simulink model "TestModel_V5_Timing_V3_2024a"  (R2024a)
settings: Solver=FixedStepAuto  StartTime=0.0  StopTime=40  FixedStep=1e-6  RelTol=1e-3
values from neighbouring files (symbols this model uses):
  par_Ctrl_FluxOffset = 0    [Param.m]
  par_Ctrl_MI = 0.99    [Param.m]
  par_Ctrl_SpdRt = 10    [Param.m]
  par_Ctrl_ThetaOffset = 0    [Param.m]
  par_IM_Frated = 50    [Param.m]
  par_IM_IratedPh = 7.9/sqrt(3)    [Param.m]
  par_IM_Lm = 0.527    [Param.m]
  par_IM_Lr = par_IM_Lm + par_IM_Llr    (= 0.5639)    [Param.m]
  par_IM_pp = 2    [Param.m]
  par_IM_Rs = 3.14    [Param.m]
  par_IM_VrmsLL = 400    [Param.m]
  par_uc_Ts = 100e-6    (= 0.0001)    [Param.m]
  pmsm = mcb.getPMSMParameters('Teknic2310P')    [mcb_pmsm_foc_sensorless_f28379d_datascript.m]
  Ts = T_pwm    (= 5e-05)    [mcb_pmsm_foc_sensorless_f28379d_datascript.m]
  Ts_motor = T_pwm/2    (= 2.5e-05)    [mcb_pmsm_foc_sensorless_f28379d_datascript.m]
undefined symbols (not defined in the file or in its folder): DiscIntNeverNeededParam, IM, par_pmsm_FluxLinkage, par_pmsm_Frated, par_pmsm_pp, par_pmsm_Vboost, par_pmsm_VrmsLL
libraries: spsOnDelayLib x24, mcbcontrolslib x12, spsTriangleGeneratorLib x4, autolibim x3, spsFirstOrderFilterLib x3, spsCurrentMeasurementLib x2, spsDCVoltageSourceLib x2, spsVoltageMeasurementLib x2, spsTwoLevelConverterLib x2, spsThreePhaseVIMeasurementLib x2, spsSeriesRLCBranchLib x1, sdolib x1
(part 3 of 3)

== matlab function TestModel_V5_Timing_V3_2024a/Open_Loop2/Estimation/MRAS_Observer ==
  data: v_alpha input; theta_est output; v_beta input; i_alpha input; i_beta input; Ts input; Rs input; Rr input; Ls input; Lr input; Lm input; Kp_SpdEst input; Ki_SpdEst input; omega_est output; e output; e_filt output; psi_r_ref_alpha output; psi_r_ref_beta output; psi_r_est_alpha1 output; psi_r_est_beta1 output; psi_est_mag1 output; psi_ref_mag1 output; psi_s_alpha1 output; psi_s_beta1 output; psi_mag_stator1 output; psi_r_est_alpha_dot1 output; psi_r_est_beta_dot1 output; Fe_Out input
function [theta_est, omega_est, e, e_filt, psi_r_ref_alpha, psi_r_ref_beta, psi_r_est_alpha1, psi_r_est_beta1, psi_est_mag1, psi_ref_mag1, psi_s_alpha1, psi_s_beta1, psi_mag_stator1, psi_r_est_alpha_dot1, psi_r_est_beta_dot1] = fcn(v_alpha, v_beta, i_alpha, i_beta, Ts, Rs, Rr, Ls, Lr, Lm, Kp_SpdEst, Ki_SpdEst, Fe_Out)

%% Motor Parameters

Tr = Lr/Rr;   % Rotor time constant
sigma = 1 - (Lm^2)/(Ls*Lr);

%% Flux Integrator Leakage Factor

wc_flux = 20;      % rad/s

%% Speed LPF Bandwidth

wc_speed = 100;   % rad/s

%% Limits

INT_LIMIT = 500;

OMEGA_MAX = 1000;
OMEGA_MIN = -1000;

FLUX_MIN = 0;
%FLUX_MIN = 0.05;

%% Persistent Variables

persistent psi_s_alpha psi_s_beta

persistent psi_r_est_alpha psi_r_est_beta

persistent omega_hat
persistent omega_filt

persistent theta_hat

persistent int_error
% persistent e_prev

if isempty(psi_s_alpha)

    psi_s_alpha = 0;
    psi_s_beta = 0;

    psi_r_est_alpha = 0;
    psi_r_est_beta = 0;

    omega_hat = 1;   % Small non-zero initial value
    omega_filt = 100;

    theta_hat = 0;

    int_error = 0;
    % e_prev = 0;

end

persistent e_filt_prv

if isempty(e_filt_prv)
    e_filt_prv = 0;
end

% if isempty(int_error)
%     int_error = 0;
% end


%% ==========================================================
%% REFERENCE MODEL
%% Voltage Model
%% ==========================================================

psi_s_alpha_dot = v_alpha - Rs*i_alpha;
psi_s_beta_dot  = v_beta  - Rs*i_beta;

% Leaky Integrator

psi_s_alpha = ...
    (1 - wc_flux*Ts)*psi_s_alpha + ...
    psi_s_alpha_dot*Ts;

psi_s_beta = ...
    (1 - wc_flux*Ts)*psi_s_beta + ...
    psi_s_beta_dot*Ts;

psi_mag_stator ...
= ...
sqrt(psi_s_alpha^2 + psi_s_beta^2);

%% Rotor Flux Reference

psi_r_ref_alpha = ...
    (Lr/Lm) * ...
    (psi_s_alpha - sigma*Ls*i_alpha);

psi_r_ref_beta = ...
    (Lr/Lm) * ...
    (psi_s_beta - sigma*Ls*i_beta);

%% ==========================================================
%% ADAPTIVE MODEL
%% ==========================================================

% omega_test= 2*pi*Fe_Out;

% psi_r_est_alpha_dot = ...
%       (Lm/Tr)*10*i_alpha ...
%     - (1/Tr)*psi_r_est_alpha ...
%     - omega_test*psi_r_est_beta;
% 
% psi_r_est_beta_dot = ...
%       (Lm/Tr)*10*i_beta ...
%     - (1/Tr)*psi_r_est_beta ...
%     + omega_test*psi_r_est_alpha;


psi_r_est_alpha_dot = ...
      (Lm/Tr)*i_alpha ...
    - (1/Tr)*psi_r_est_alpha ...
    - omega_filt*psi_r_est_beta;

psi_r_est_beta_dot = ...
      (Lm/Tr)*i_beta ...
    - (1/Tr)*psi_r_est_beta ...
    + omega_filt*psi_r_est_alpha;

psi_r_est_alpha = ...
    psi_r_est_alpha + ...
    psi_r_est_alpha_dot*Ts;

psi_r_est_beta = ...
    psi_r_est_beta + ...
    psi_r_est_beta_dot*Ts;



%% ==========================================================
%% ADAPTATION ERROR
%% ==========================================================

flux_sq = psi_r_est_alpha^2 + psi_r_est_beta^2 + 1e-6;

e =...
(psi_r_ref_alpha*psi_r_est_beta ...
- psi_r_ref_beta*psi_r_est_alpha)/flux_sq;

% e = ...
%       psi_r_ref_alpha * psi_r_est_beta ...
%     - psi_r_ref_beta  * psi_r_est_alpha;

%% ==========================================================
%% FLUX MAGNITUDE CHECK
%% ==========================================================

psi_est_mag = sqrt( ...
    psi_r_est_alpha^2 + ...
    psi_r_est_beta^2 );

psi_ref_mag = sqrt( ...
    psi_r_ref_alpha^2 + ...
    psi_r_ref_beta^2 );

if psi_est_mag < FLUX_MIN

    omega_hat = 0;
    omega_filt = 0;

else




    %% ======================================================
    %% PI ADAPTATION
    %% ======================================================


wc_e = 20;

e_filt_prv = e_filt_prv + ...
         wc_e*Ts*(e-e_filt_prv);


    int_error = int_error + e_filt_prv*Ts;

    if int_error > INT_LIMIT
        int_error = INT_LIMIT;
    elseif int_error < -INT_LIMIT
        int_error = -INT_LIMIT;
    end

    %% Incremental PI

    % domega = ...
    %       Kp_SpdEst*(e_filt_prv - e_prev) ...
    %     + Ki_SpdEst*e_filt_prv*Ts;
    % 
    % omega_hat = omega_hat + domega;

    %% Continuous PI

    % int_error = int_error + e_filt_prv*Ts;

omega_hat = ...
      Kp_SpdEst*e_filt_prv ...
    + Ki_SpdEst*int_error;

    %% Speed Limit

    if omega_hat > OMEGA_MAX
        omega_hat = OMEGA_MAX;
    elseif omega_hat < OMEGA_MIN
        omega_hat = OMEGA_MIN;
    end

    %% Speed LPF

    omega_filt = ...
        omega_filt + ...
        wc_speed*Ts*(omega_hat - omega_filt);

end

%% Save Previous Error

% e_prev = e_filt_prv;

%% ==========================================================
%% THETA ESTIMATION
%% ==========================================================


theta_hat = ...
atan2(psi_r_est_beta,...
      psi_r_est_alpha);

% theta_hat = theta_hat + omega_filt*Ts;
% 
% theta_hat = mod(theta_hat,2*pi);

%% Outputs

theta_est = theta_hat;
omega_est = omega_filt;
e_filt=e_filt_prv;
psi_r_est_alpha1=psi_r_est_alpha;
psi_r_est_beta1=psi_r_est_beta;
psi_est_mag1=psi_est_mag;
psi_ref_mag1=psi_ref_mag;
psi_s_alpha1=psi_s_alpha;
psi_s_beta1=psi_s_beta;
psi_mag_stator1=psi_mag_stator;
psi_r_est_alpha_dot1=psi_r_est_alpha_dot;
psi_r_est_beta_dot1=psi_r_est_beta_dot;

end


%%

% %% Initialize States
% 
% % psi_ref = [0; 0];   % reference flux (alpha, beta)
% % psi_est = [0; 0];   % estimated flux
% % 
% % omega_est = 0;
% % theta_est = 0;
% % 
% % int_error = 0;
% 
% persistent psi_s_alpha psi_s_beta
% persistent psi_r_est_alpha psi_r_est_beta
% persistent omega_hat
% persistent theta_hat
% persistent int_error
% 
% if isempty(psi_s_alpha)
%     psi_s_alpha = 0;
%     psi_s_beta = 0;
%     psi_r_est_alpha = 0;
%     psi_r_est_beta = 0;
%     omega_hat = 0;
%     theta_hat = 0;
%     int_error = 0;
% end
% 
% %% Reference Model
% 
% % Inputs: Valpha, Vbeta, Ialpha, Ibeta
% 
% % psi_ref_dot = [v_alpha; v_beta] - Rs * [i_alpha; i_beta];
% % psi_ref = psi_ref + psi_ref_dot * Ts;
% 
% psi_s_alpha_dot = v_alpha - Rs * i_alpha;
% psi_s_beta_dot =  v_beta  - Rs * i_beta;
% psi_s_alpha = psi_s_alpha + psi_s_alpha_dot * Ts;
% psi_s_beta  = psi_s_beta + psi_s_beta_dot * Ts;
% 
% %% Rotor Flux Reference
% 
% psi_r_ref_alpha = (Lr/Lm) * (psi_s_alpha - sigma*Ls*i_alpha);
% 
% psi_r_ref_beta = (Lr/Lm) * (psi_s_beta - sigma*Ls*i_beta);
% 
% %% Adaptive Model 
% 
% % psi_est_dot = (Lm/Tr) * [i_alpha; i_beta] ...
% %               - (1/Tr) * psi_est ...
% %               - omega_est * [0 -1; 1 0] * psi_est;
% % 
% % psi_est = psi_est + psi_est_dot * Ts;
% 
% psi_r_est_alpha_dot = (Lm/Tr)*i_alpha - (1/Tr)*psi_r_est_alpha + omega_hat*psi_r_est_beta;
% 
% psi_r_est_beta_dot = (Lm/Tr)*i_beta - (1/Tr)*psi_r_est_beta - omega_hat*psi_r_est_alpha;
% 
% psi_r_est_alpha = psi_r_est_alpha + psi_r_est_alpha_dot*Ts;
% 
% psi_r_est_beta = psi_r_est_beta + psi_r_est_beta_dot*Ts;
% 
% %% Error Calculation
% 
% % e = psi_ref(1) * psi_est(2) - psi_ref(2) * psi_est(1);    % Error Calculation
% 
% e = psi_r_ref_alpha*psi_r_est_beta - psi_r_ref_beta *psi_r_est_alpha;
% 
% %% Speed Estimation
% 
% int_error = int_error + e * Ts;
% 
% % Anti-windup
% INT_LIMIT = 500;
% 
% if int_error > INT_LIMIT
%     int_error = INT_LIMIT;
% elseif int_error < -INT_LIMIT
%     int_error = -INT_LIMIT;
% end
% 
% omega_hat = Kp_SpdEst * e + Ki_SpdEst * int_error;
% 
% %Speed Limit
% 
% OMEGA_MAX = 1000;
% 
% if omega_hat > OMEGA_MAX
%     omega_hat = OMEGA_MAX;
% elseif omega_hat < -OMEGA_MAX
%     omega_hat = -OMEGA_MAX;
% end
% 
% 
% %% Angle Update
% 
% % theta_est = theta_est + omega_est * Ts;
% 
% theta_hat = theta_hat + omega_hat*Ts;
% %% Wrap Angle
% 
% %theta_est_obs = mod(theta_est, 2*pi);
% 
% theta_hat = mod(theta_hat,2*pi);
% 
% %% Outputs
% 
% theta_est = theta_hat;
% 
% omega_est = omega_hat;
% 
% end

== matlab function TestModel_V5_Timing_V3_2024a/Open_Loop2/Subsystem1/MATLAB Function ==
  data: fe input; Vs output; Vs1 input; V_Boost input
function Vs = fcn(fe,Vs1,V_Boost)
%#codegen

if fe<6
    Vs=Vs1+V_Boost;
else
    Vs=Vs1;
end
end

== matlab function TestModel_V5_Timing_V3_2024a/Open_Loop2/Subsystem1/MATLAB Function5 ==
  data: u input; y output; data input
%FileName: Ramp1
%Description: Function to ramp input u1 from output value u2. 
%Inputs: Any Signal Value
%Output: Ramp of input signal until the input value
%Created by: Devi Cheerla
%Created on: 21-08-2024
%Version no: 0.1

function y = ramp1(u, data)
u1=u;
u2=data;
dy=0.001*4;
persistent yp;
if isempty(yp)
    yp=0;
elseif (yp==yp && yp~=u2)
    yp=u2;
else
end
diff = u1-yp;

if diff>0
    y=yp+dy;
elseif diff<0
    y=yp-dy;
else
    y=yp;
end
yp=y;

end

== matlab function TestModel_V5_Timing_V3_2024a/MATLAB Function2 ==
  data: V_Alpha input; V_Beta input; Flt_Out input; y1 output; y2 output; PWM_En input; GtDrEn input
function [y1,y2] = fcn(V_Alpha, V_Beta, Flt_Out, PWM_En, GtDrEn)
%#codegen
if Flt_Out == 0 && PWM_En==1 && GtDrEn==1
    y1= V_Alpha;
    y2= V_Beta;
else
    y1=0;
    y2=0;
end
end

== matlab function TestModel_V5_Timing_V3_2024a/MATLAB Function4 ==
  data: RmsCalEn output; Fe2 input; Fe1 input
function RmsCalEn = fcn(Fe2, Fe1)

err=Fe2-Fe1;
for err>0
    
if Fe1==0.95*Fe2
    RmsCalEn=1;
else
    RmsCalEn=0;
end
end

== matlab function TestModel_V5_Timing_V3_2024a/Open_Loop2/Estimation/MRAS_Observer1 ==
  data: v_alpha input; theta_est output; v_beta input; i_alpha input; i_beta input; Ts input; Rs input; Rr input; Ls input; Lr input; Lm input; Kp_SpdEst input; Ki_SpdEst input; omega_est output
function [theta_est, omega_est] = fcn(v_alpha, v_beta, i_alpha, i_beta, Ts, Rs, Rr, Ls, Lr, Lm, Kp_SpdEst, Ki_SpdEst)

Tr=Lr/Rr;    % Rotor time constant
sigma = 1 - (Lm^2)/(Ls*Lr);

%% Initialize States

% psi_ref = [0; 0];   % reference flux (alpha, beta)
% psi_est = [0; 0];   % estimated flux
% 
% omega_est = 0;
% theta_est = 0;
% 
% int_error = 0;

persistent psi_s_alpha psi_s_beta
persistent psi_r_est_alpha psi_r_est_beta
persistent omega_hat
persistent theta_hat
persistent int_error

if isempty(psi_s_alpha)
    psi_s_alpha = 0;
    psi_s_beta = 0;
    psi_r_est_alpha = 0;
    psi_r_est_beta = 0;
    omega_hat = 0;
    theta_hat = 0;
    int_error = 0;
end

%% Reference Model

% Inputs: Valpha, Vbeta, Ialpha, Ibeta

% psi_ref_dot = [v_alpha; v_beta] - Rs * [i_alpha; i_beta];
% psi_ref = psi_ref + psi_ref_dot * Ts;

psi_s_alpha_dot = v_alpha - Rs * i_alpha;
psi_s_beta_dot =  v_beta  - Rs * i_beta;
psi_s_alpha = psi_s_alpha + psi_s_alpha_dot * Ts;
psi_s_beta  = psi_s_beta + psi_s_beta_dot * Ts;

%% Rotor Flux Reference

psi_r_ref_alpha = (Lr/Lm) * (psi_s_alpha - sigma*Ls*i_alpha);

psi_r_ref_beta = (Lr/Lm) * (psi_s_beta - sigma*Ls*i_beta);

%% Adaptive Model 

% psi_est_dot = (Lm/Tr) * [i_alpha; i_beta] ...
%               - (1/Tr) * psi_est ...
%               - omega_est * [0 -1; 1 0] * psi_est;
% 
% psi_est = psi_est + psi_est_dot * Ts;

psi_r_est_alpha_dot = (Lm/Tr)*i_alpha - (1/Tr)*psi_r_est_alpha + omega_hat*psi_r_est_beta;

psi_r_est_beta_dot = (Lm/Tr)*i_beta - (1/Tr)*psi_r_est_beta - omega_hat*psi_r_est_alpha;

psi_r_est_alpha = psi_r_est_alpha + psi_r_est_alpha_dot*Ts;

psi_r_est_beta = psi_r_est_beta + psi_r_est_beta_dot*Ts;

%% Error Calculation

% e = psi_ref(1) * psi_est(2) - psi_ref(2) * psi_est(1);    % Error Calculation

e = psi_r_ref_alpha*psi_r_est_beta - psi_r_ref_beta *psi_r_est_alpha;

%% Speed Estimation

int_error = int_error + e * Ts;

% Anti-windup
INT_LIMIT = 500;

if int_error > INT_LIMIT
    int_error = INT_LIMIT;
elseif int_error < -INT_LIMIT
    int_error = -INT_LIMIT;
end

omega_hat = Kp_SpdEst * e + Ki_SpdEst * int_error;

%Speed Limit

OMEGA_MAX = 1000;

if omega_hat > OMEGA_MAX
    omega_hat = OMEGA_MAX;
elseif omega_hat < -OMEGA_MAX
    omega_hat = -OMEGA_MAX;
end


%% Angle Update

% theta_est = theta_est + omega_est * Ts;

theta_hat = theta_hat + omega_hat*Ts;
%% Wrap Angle

%theta_est_obs = mod(theta_est, 2*pi);

theta_hat = mod(theta_hat,2*pi);

%% Outputs

theta_est = theta_hat;

omega_est = omega_hat;

end

== matlab function TestModel_V5_Timing_V3_2024a/Open_Loop2/MATLAB Function1 ==
  data: u1 input; y1 output; u2 input; Ts input; y2 output
function [y1,y2] = LPF(u1,u2,Ts)

persistent y1_prev y2_prev

fc = 80;          % Hz
wc = 2*pi*fc;

if isempty(y1_prev)
    y1_prev = 0;
end

if isempty(y2_prev)
    y2_prev = 0;
end

alpha = wc*Ts;
beta  = wc*Ts;

y1 = y1_prev + alpha*(u1 - y1_prev);
y2 = y2_prev + beta*(u2 - y2_prev);

y1_prev = y1;
y2_prev = y2;

end

== matlab function TestModel_V5_Timing_V3_2024a/Open_Loop/MATLAB Function ==
  data: fe input; Vs output; Vs1 input; V_Boost input
function Vs = fcn(fe,Vs1,V_Boost)
%#codegen

% if fe<6
%     Vs=Vs1+V_Boost;
% else
%     Vs=Vs1;
% end

if fe<=0
    Vs = 0;
elseif fe>0 || fe<50
    Vs = V_Boost + (400-V_Boost)*fe/50;  %    V_Boost(1+(Vs1/V_Boost)-(fe/50))
else
    Vs= 400;
end

end

== matlab function TestModel_V5_Timing_V3_2024a/Open_Loop/Subsystem/MATLAB Function5 ==
  data: u input; y output; data input
%FileName: Ramp1
%Description: Function to ramp input u1 from output value u2. 
%Inputs: Any Signal Value
%Output: Ramp of input signal until the input value
%Created by: Devi Cheerla
%Created on: 21-08-2024
%Version no: 0.1

function y = ramp1(u, data)
u1=u;
u2=data;
dy=0.001*4;
persistent yp;
if isempty(yp)
    yp=0;
elseif (yp==yp && yp~=u2)
    yp=u2;
else
end
diff = u1-yp;

if diff>0
    y=yp+dy;
elseif diff<0
    y=yp-dy;
else
    y=yp;
end
yp=y;

end

== matlab function TestModel_V5_Timing_V3_2024a/Open_Loop2/Subsystem1/MATLAB Function1 ==
  data: speed_cmd input; y output; ramp_rate input; Ts input
%FileName: Ramp1
%Description: Function to ramp input u1 from output value u2. 
%Inputs: Any Signal Value
%Output: Ramp of input signal until the input value
%Created by: Devi Cheerla
%Created on: 21-08-2024
%Version no: 0.1

% function y = ramp1(u, data)
% u1=u;
% u2=data;
% dy=0.001*4;
% persistent yp;
% if isempty(yp)
%     yp=0;
% elseif (yp==yp && yp~=u2)
%     yp=u2;
% else
% end
% diff = u1-yp;
% 
% if diff>0
%     y=yp+dy;
% elseif diff<0
%     y=yp-dy;
% else
%     y=yp;
% end
% yp=y;
% 
% end


function y = speed_ramp(speed_cmd,ramp_rate,Ts)

persistent speed_ref

%Ts = 1e-6;
%Ts = 10e-3;

dN = ramp_rate * Ts;

if isempty(speed_ref)
    speed_ref = 0;
end

err = speed_cmd - speed_ref;

if abs(err) <= dN
    speed_ref = speed_cmd;
elseif err > 0
    speed_ref = speed_ref + dN;
else
    speed_ref = speed_ref - dN;
end

y = speed_ref;

end

== matlab function TestModel_V5_Timing_V3_2024a/Open_Loop2/MATLAB Function2 ==
  data: speed_cmd input; y output; RampUpRate input; RampDownRate input; Ts input
%FileName: Ramp1
%Description: Function to ramp input u1 from output value u2. 
%Inputs: Any Signal Value
%Output: Ramp of input signal until the input value
%Created by: Devi Cheerla
%Created on: 21-08-2024
%Version no: 0.1

% function y = ramp1(u, data)
% u1=u;
% u2=data;
% dy=0.001*4;
% persistent yp;
% if isempty(yp)
%     yp=0;
% elseif (yp==yp && yp~=u2)
%     yp=u2;
% else
% end
% diff = u1-yp;
% 
% if diff>0
%     y=yp+dy;
% elseif diff<0
%     y=yp-dy;
% else
%     y=yp;
% end
% yp=y;
% 
% end


% function y = speed_ramp(speed_cmd,ramp_rate,Ts)
% 
% persistent speed_ref
% 
% % Ts = 1e-6;
% 
% dN = ramp_rate * Ts;
% 
% if isempty(speed_ref)
%     speed_ref = 0;
% end
% 
% err = speed_cmd - speed_ref;
% 
% if abs(err) <= dN
%     speed_ref = speed_cmd;
% elseif err > 0
%     speed_ref = speed_ref + dN;
% else
%     speed_ref = speed_ref - dN;
% end
% 
% y = speed_ref;
% 
% end

function y = speed_ramp(speed_cmd, RampUpRate, RampDownRate, Ts )

persistent speed_ref

% Ts = 1e-3;
% 
% RampUpRate   = 25;
% RampDownRate = 100;

if isempty(speed_ref)
    speed_ref = 0;
end

err = speed_cmd - speed_ref;

if err > 0

    dN = RampUpRate * Ts;

    if err <= dN
        speed_ref = speed_cmd;
    else
        speed_ref = speed_ref + dN;
    end

elseif err < 0

    dN = RampDownRate * Ts;

    if abs(err) <= dN
        speed_ref = speed_cmd;
    else
        speed_ref = speed_ref - dN;
    end

end

y = speed_ref;

end

== matlab function TestModel_V5_Timing_V3_2024a/Open_Loop2/Subsystem1/MATLAB Function3 ==
  data: u input; y output; data input
%FileName: Ramp1
%Description: Function to ramp input u1 from output value u2. 
%Inputs: Any Signal Value
%Output: Ramp of input signal until the input value
%Created by: Devi Cheerla
%Created on: 21-08-2024
%Version no: 0.1

function y = ramp1(u, data)
u1=u;
u2=data;
dy=0.001*4;
persistent yp;
if isempty(yp)
    yp=0;
elseif (yp==yp && yp~=u2)
    yp=u2;
else
end
diff = u1-yp;

if diff>0
    y=yp+dy;
elseif diff<0
    y=yp-dy;
else
    y=yp;
end
yp=y;

end

== matlab function TestModel_V5_Timing_V3_2024a/Open_Loop2/Estimation/EBE_Observer ==
  data: i_alpha_hat output; i_beta_hat output; e_alpha_hat output; e_beta_hat output; v_alpha input; v_beta input; i_alpha_meas input; i_beta_meas input; Ts input; Rs input; L input; ki input; ke input
function [i_alpha_hat, i_beta_hat, e_alpha_hat, e_beta_hat] = ...
    ebe_step(v_alpha, v_beta, i_alpha_meas, i_beta_meas, Ts, Rs, L, ki, ke)

%#codegen
persistent i_alpha_hat_z i_beta_hat_z e_alpha_hat_z e_beta_hat_z
if isempty(i_alpha_hat_z)
    i_alpha_hat_z = i_alpha_meas;  % init at first sample
    i_beta_hat_z  = i_beta_meas;
    e_alpha_hat_z = 0.0;
    e_beta_hat_z  = 0.0;
end

% Errors
i_alpha_tilde = i_alpha_meas - i_alpha_hat_z;
i_beta_tilde  = i_beta_meas  - i_beta_hat_z;

% Current observer dynamics (discrete Euler)
di_alpha_hat = (1/L)*(v_alpha - Rs*i_alpha_hat_z - e_alpha_hat_z) + ki*i_alpha_tilde;
di_beta_hat  = (1/L)*(v_beta  - Rs*i_beta_hat_z  - e_beta_hat_z)  + ki*i_beta_tilde;

i_alpha_hat_next = i_alpha_hat_z + Ts*di_alpha_hat;
i_beta_hat_next  = i_beta_hat_z  + Ts*di_beta_hat;

% Back-EMF observer dynamics (discrete Euler)
de_alpha_hat = ke * i_alpha_tilde;
de_beta_hat  = ke * i_beta_tilde;

e_alpha_hat_next = e_alpha_hat_z + Ts*de_alpha_hat;
e_beta_hat_next  = e_beta_hat_z  + Ts*de_beta_hat;

% Optional: saturation on e_hat to avoid wind-up
E_MAX = 1e4; % set based on machine
e_alpha_hat_next = min(max(e_alpha_hat_next, -E_MAX), E_MAX);
e_beta_hat_next  = min(max(e_beta_hat_next,  -E_MAX),  E_MAX);

% Update state
i_alpha_hat_z = i_alpha_hat_next;
i_beta_hat_z  = i_beta_hat_next;
e_alpha_hat_z = e_alpha_hat_next;
e_beta_hat_z  = e_beta_hat_next;

% Outputs
i_alpha_hat = i_alpha_hat_z;
i_beta_hat  = i_beta_hat_z;
e_alpha_hat = e_alpha_hat_z;
e_beta_hat  = e_beta_hat_z;
end

== matlab function TestModel_V5_Timing_V3_2024a/Open_Loop2/MATLAB Function4 ==
  data: fe input; Vs output; Vs1 input; V_Boost input
function Vs = fcn(fe,Vs1,V_Boost)
%#codegen

% if fe<6
%     Vs=Vs1+V_Boost;
% else
%     Vs=Vs1;
% end

if fe<=0
    Vs = 0;
elseif fe>0 || fe<50
    Vs = V_Boost + (400-V_Boost)*fe/50;  %    V_Boost(1+(Vs1/V_Boost)-(fe/50))
else
    Vs= 400;
end

end

== matlab function TestModel_V5_Timing_V3_2024a/Open_Loop2/RotorFluxEstimation ==
  data: psi_d_Rot output; psi_q_Rot output; IdSta input; IqSta input; IdRot input; IqRot input; Lm input; Lr input; psi_mag output; Is output
function [psi_d_Rot, psi_q_Rot, psi_mag, Is] = ...
    ebe_step(IdSta, IqSta, IdRot,IqRot, Lm, Lr)

psi_d_Rot = Lr*IdRot + Lm*IdSta;
psi_q_Rot = Lr*IqRot + Lm*IqSta;

psi_mag = sqrt(psi_d_Rot.^2 + psi_q_Rot.^2);
Is = sqrt(IdSta.^2 + IqSta.^2);

end

== matlab function TestModel_V5_Timing_V3_2024a/Open_Loop2/Subsystem/MATLAB Function ==
  data: StartPulse input; PreMag_En output
function PreMag_En = PreMagState(StartPulse)

persistent timer active

Ts = 1e-6;
PreMagTime = 0.2;    % 200 ms

if isempty(timer)
    timer = 0;
    active = 0;
end

if isempty(active)
    timer = 0;
    active = 0;
end

if StartPulse
    %timer = 0;
    active = 1;
    timer = timer + Ts;
    if timer >= PreMagTime
        active = 0;
    end
end

% if active
% 
%     timer = timer + Ts;
% 
%     if timer >= PreMagTime
%         active = 0;
%     end
% 
% end

% if StartPulse
%     timer = 0;
%     active = 1;
% end
% 
% if active
% 
%     timer = timer + Ts;
% 
%     if timer >= PreMagTime
%         active = 0;
%     end
% 
% end

PreMag_En = active;
end

== matlab function TestModel_V5_Timing_V3_2024a/Open_Loop2/Subsystem/MATLAB Function1 ==
  data: PreMag_En input; Fe_Out output; Fe_Ramp input
function Fe_Out = PreMagState(PreMag_En, Fe_Ramp)

if PreMag_En > 0 && PreMag_En < 2
    Fe_Out = 1;
else
    Fe_Out = Fe_Ramp;
end

== matlab function TestModel_V5_Timing_V3_2024a/Open_Loop2/Subsystem/MATLAB Function2 ==
  data: speed_cmd input; y output; RampUpRate input; RampDownRate input; Ts input
%FileName: Ramp1
%Description: Function to ramp input u1 from output value u2. 
%Inputs: Any Signal Value
%Output: Ramp of input signal until the input value
%Created by: Devi Cheerla
%Created on: 21-08-2024
%Version no: 0.1

% function y = ramp1(u, data)
% u1=u;
% u2=data;
% dy=0.001*4;
% persistent yp;
% if isempty(yp)
%     yp=0;
% elseif (yp==yp && yp~=u2)
%     yp=u2;
% else
% end
% diff = u1-yp;
% 
% if diff>0
%     y=yp+dy;
% elseif diff<0
%     y=yp-dy;
% else
%     y=yp;
% end
% yp=y;
% 
% end


% function y = speed_ramp(speed_cmd,ramp_rate,Ts)
% 
% persistent speed_ref
% 
% % Ts = 1e-6;
% 
% dN = ramp_rate * Ts;
% 
% if isempty(speed_ref)
%     speed_ref = 0;
% end
% 
% err = speed_cmd - speed_ref;
% 
% if abs(err) <= dN
%     speed_ref = speed_cmd;
% elseif err > 0
%     speed_ref = speed_ref + dN;
% else
%     speed_ref = speed_ref - dN;
% end
% 
% y = speed_ref;
% 
% end

function y = speed_ramp(speed_cmd, RampUpRate, RampDownRate, Ts )

persistent speed_ref

% Ts = 1e-3;
% 
% RampUpRate   = 25;
% RampDownRate = 100;

if isempty(speed_ref)
    speed_ref = 0;
end

err = speed_cmd - speed_ref;

if err > 0

    dN = RampUpRate * Ts;

    if err <= dN
        speed_ref = speed_cmd;
    else
        speed_ref = speed_ref + dN;
    end

elseif err < 0

    dN = RampDownRate * Ts;

    if abs(err) <= dN
        speed_ref = speed_cmd;
    else
        speed_ref = speed_ref - dN;
    end

end

y = speed_ref;

end

== matlab function TestModel_V5_Timing_V3_2024a/Open_Loop/Subsystem/MATLAB Function1 ==
  data: speed_cmd input; y output; ramp_rate input; Ts input
%FileName: Ramp1
%Description: Function to ramp input u1 from output value u2. 
%Inputs: Any Signal Value
%Output: Ramp of input signal until the input value
%Created by: Devi Cheerla
%Created on: 21-08-2024
%Version no: 0.1

% function y = ramp1(u, data)
% u1=u;
% u2=data;
% dy=0.001*4;
% persistent yp;
% if isempty(yp)
%     yp=0;
% elseif (yp==yp && yp~=u2)
%     yp=u2;
% else
% end
% diff = u1-yp;
% 
% if diff>0
%     y=yp+dy;
% elseif diff<0
%     y=yp-dy;
% else
%     y=yp;
% end
% yp=y;
% 
% end


function y = speed_ramp(speed_cmd,ramp_rate,Ts)

persistent speed_ref

%Ts = 1e-6;
%Ts = 10e-3;

dN = ramp_rate * Ts;

if isempty(speed_ref)
    speed_ref = 0;
end

err = speed_cmd - speed_ref;

if abs(err) <= dN
    speed_ref = speed_cmd;
elseif err > 0
    speed_ref = speed_ref + dN;
else
    speed_ref = speed_ref - dN;
end

y = speed_ref;

end

== matlab function TestModel_V5_Timing_V3_2024a/Subsystem3/Estimation/MRAS_Observer ==
  data: v_alpha input; theta_est output; v_beta input; i_alpha input; i_beta input; Ts input; Rs input; Rr input; Ls input; Lr input; Lm input; Kp_SpdEst input; Ki_SpdEst input; omega_est output
function [theta_est, omega_est] = fcn(v_alpha, v_beta, i_alpha, i_beta, Ts, Rs, Rr, Ls, Lr, Lm, Kp_SpdEst, Ki_SpdEst)

Tr=Lr/Rr;    % Rotor time constant
sigma = 1 - (Lm^2)/(Ls*Lr);

%% Initialize States

% psi_ref = [0; 0];   % reference flux (alpha, beta)
% psi_est = [0; 0];   % estimated flux
% 
% omega_est = 0;
% theta_est = 0;
% 
% int_error = 0;

persistent psi_s_alpha psi_s_beta
persistent psi_r_est_alpha psi_r_est_beta
persistent omega_hat
persistent theta_hat
persistent int_error

if isempty(psi_s_alpha)
    psi_s_alpha = 0;
    psi_s_beta = 0;
    psi_r_est_alpha = 0;
    psi_r_est_beta = 0;
    omega_hat = 0;
    theta_hat = 0;
    int_error = 0;
end

%% Reference Model

% Inputs: Valpha, Vbeta, Ialpha, Ibeta

% psi_ref_dot = [v_alpha; v_beta] - Rs * [i_alpha; i_beta];
% psi_ref = psi_ref + psi_ref_dot * Ts;

psi_s_alpha_dot = v_alpha - Rs * i_alpha;
psi_s_beta_dot =  v_beta  - Rs * i_beta;
psi_s_alpha = psi_s_alpha + psi_s_alpha_dot * Ts;
psi_s_beta  = psi_s_beta + psi_s_beta_dot * Ts;

%% Rotor Flux Reference

psi_r_ref_alpha = (Lr/Lm) * (psi_s_alpha - sigma*Ls*i_alpha);

psi_r_ref_beta = (Lr/Lm) * (psi_s_beta - sigma*Ls*i_beta);

%% Adaptive Model 

% psi_est_dot = (Lm/Tr) * [i_alpha; i_beta] ...
%               - (1/Tr) * psi_est ...
%               - omega_est * [0 -1; 1 0] * psi_est;
% 
% psi_est = psi_est + psi_est_dot * Ts;

psi_r_est_alpha_dot = (Lm/Tr)*i_alpha - (1/Tr)*psi_r_est_alpha + omega_hat*psi_r_est_beta;

psi_r_est_beta_dot = (Lm/Tr)*i_beta - (1/Tr)*psi_r_est_beta - omega_hat*psi_r_est_alpha;

psi_r_est_alpha = psi_r_est_alpha + psi_r_est_alpha_dot*Ts;

psi_r_est_beta = psi_r_est_beta + psi_r_est_beta_dot*Ts;

%% Error Calculation

% e = psi_ref(1) * psi_est(2) - psi_ref(2) * psi_est(1);    % Error Calculation

e = psi_r_ref_alpha*psi_r_est_beta - psi_r_ref_beta *psi_r_est_alpha;

%% Speed Estimation

int_error = int_error + e * Ts;

% Anti-windup
INT_LIMIT = 500;

if int_error > INT_LIMIT
    int_error = INT_LIMIT;
elseif int_error < -INT_LIMIT
    int_error = -INT_LIMIT;
end

omega_hat = Kp_SpdEst * e + Ki_SpdEst * int_error;

%Speed Limit

OMEGA_MAX = 1000;

if omega_hat > OMEGA_MAX
    omega_hat = OMEGA_MAX;
elseif omega_hat < -OMEGA_MAX
    omega_hat = -OMEGA_MAX;
end


%% Angle Update

% theta_est = theta_est + omega_est * Ts;

theta_hat = theta_hat + omega_hat*Ts;
%% Wrap Angle

%theta_est_obs = mod(theta_est, 2*pi);

theta_hat = mod(theta_hat,2*pi);

%% Outputs

theta_est = theta_hat;

omega_est = omega_hat;

end

== matlab function TestModel_V5_Timing_V3_2024a/Open_Loop2/Subsystem/MATLAB Function4 ==
  data: PreMag_En input; fe input; Vs output; Vs1 input; V_Boost input
function Vs = fcn(PreMag_En, fe,Vs1,V_Boost)
%#codegen

% if fe<6
%     Vs=Vs1+V_Boost;
% else
%     Vs=Vs1;
% end
if PreMag_En == 1
    Vs= V_Boost;
else
    Vs= V_Boost + (400-V_Boost)*fe/50;  %    V_Boost(1+(Vs1/V_Boost)-(fe/50)
end

end

== matlab function TestModel_V5_Timing_V3_2024a/RMS/down ==
  data: u1 input; y output; u2 input
function y = fcn(u1,u2)
if u1>u2
    y = 1;
else
    y = 0;
end
end

== matlab function TestModel_V5_Timing_V3_2024a/RMS/max_finder ==
  data: u1 input; y output; u2 input; u3 input
function y = max(u1,u2, u3)
if u1>u2
    y = u1;
elseif u2>u1 
    y = u2;
else 
    y=u3;
end
end

== matlab function TestModel_V5_Timing_V3_2024a/Open_Loop1/MATLAB Function5 ==
  data: u input; y output; data input
%FileName: Ramp1
%Description: Function to ramp input u1 from output value u2. 
%Inputs: Any Signal Value
%Output: Ramp of input signal until the input value
%Created by: Devi Cheerla
%Created on: 21-08-2024
%Version no: 0.1

function y = ramp1(u, data)
u1=u;
u2=data;
dy=0.001*4;
persistent yp;
if isempty(yp)
    yp=0;
elseif (yp==yp && yp~=u2)
    yp=u2;
else
end
diff = u1-yp;

if diff>0
    y=yp+dy;
elseif diff<0
    y=yp-dy;
else
    y=yp;
end
yp=y;

end

== matlab function TestModel_V5_Timing_V3_2024a/Open_Loop1/Inverse_Clark1 ==
  data: v_alpha input; v_a output; v_beta input; v_b output; v_c output
function [v_a, v_b, v_c] = fcn(v_alpha,v_beta)

v_a = v_alpha;
v_b = (-1/2)*v_alpha + (sqrt(3)/2)*v_beta;
v_c = (-1/2)*v_alpha - (sqrt(3)/2)*v_beta;

end

== matlab function TestModel_V5_Timing_V3_2024a/MATLAB Function ==
  data: V_Ph input; va output; vb output; vc output; t input
function [va,vb,vc] = fcn(V_Ph,t)

f = 50;
Vpk = sqrt(2)*V_Ph;


% for t=0:Ts:1/f
    va = Vpk*sin(2*pi*f*t);
    vb = Vpk*sin(2*pi*f*t - 2*pi/3);
    vc = Vpk*sin(2*pi*f*t + 2*pi/3);
% end
end

== matlab function TestModel_V5_Timing_V3_2024a/Open_Loop/MATLAB Function2 ==
  data: speed_cmd input; y output; RampUpRate input; RampDownRate input; Ts input
%FileName: Ramp1
%Description: Function to ramp input u1 from output value u2. 
%Inputs: Any Signal Value
%Output: Ramp of input signal until the input value
%Created by: Devi Cheerla
%Created on: 21-08-2024
%Version no: 0.1

% function y = ramp1(u, data)
% u1=u;
% u2=data;
% dy=0.001*4;
% persistent yp;
% if isempty(yp)
%     yp=0;
% elseif (yp==yp && yp~=u2)
%     yp=u2;
% else
% end
% diff = u1-yp;
% 
% if diff>0
%     y=yp+dy;
% elseif diff<0
%     y=yp-dy;
% else
%     y=yp;
% end
% yp=y;
% 
% end


% function y = speed_ramp(speed_cmd,ramp_rate,Ts)
% 
% persistent speed_ref
% 
% % Ts = 1e-6;
% 
% dN = ramp_rate * Ts;
% 
% if isempty(speed_ref)
%     speed_ref = 0;
% end
% 
% err = speed_cmd - speed_ref;
% 
% if abs(err) <= dN
%     speed_ref = speed_cmd;
% elseif err > 0
%     speed_ref = speed_ref + dN;
% else
%     speed_ref = speed_ref - dN;
% end
% 
% y = speed_ref;
% 
% end

function y = speed_ramp(speed_cmd, RampUpRate, RampDownRate, Ts )

persistent speed_ref

% Ts = 1e-3;
% 
% RampUpRate   = 25;
% RampDownRate = 100;

if isempty(speed_ref)
    speed_ref = 0;
end

err = speed_cmd - speed_ref;

if err > 0

    dN = RampUpRate * Ts;

    if err <= dN
        speed_ref = speed_cmd;
    else
        speed_ref = speed_ref + dN;
    end

elseif err < 0

    dN = RampDownRate * Ts;

    if abs(err) <= dN
        speed_ref = speed_cmd;
    else
        speed_ref = speed_ref - dN;
    end

end

y = speed_ref;

end

== matlab function TestModel_V5_Timing_V3_2024a/Subsystem3/Estimation/EBE_Observer ==
  data: i_alpha_hat output; i_beta_hat output; e_alpha_hat output; e_beta_hat output; v_alpha input; v_beta input; i_alpha_meas input; i_beta_meas input; Ts input; Rs input; L input; ki input; ke input
function [i_alpha_hat, i_beta_hat, e_alpha_hat, e_beta_hat] = ...
    ebe_step(v_alpha, v_beta, i_alpha_meas, i_beta_meas, Ts, Rs, L, ki, ke)

%#codegen
persistent i_alpha_hat_z i_beta_hat_z e_alpha_hat_z e_beta_hat_z
if isempty(i_alpha_hat_z)
    i_alpha_hat_z = i_alpha_meas;  % init at first sample
    i_beta_hat_z  = i_beta_meas;
    e_alpha_hat_z = 0.0;
    e_beta_hat_z  = 0.0;
end

% Errors
i_alpha_tilde = i_alpha_meas - i_alpha_hat_z;
i_beta_tilde  = i_beta_meas  - i_beta_hat_z;

% Current observer dynamics (discrete Euler)
di_alpha_hat = (1/L)*(v_alpha - Rs*i_alpha_hat_z - e_alpha_hat_z) + ki*i_alpha_tilde;
di_beta_hat  = (1/L)*(v_beta  - Rs*i_beta_hat_z  - e_beta_hat_z)  + ki*i_beta_tilde;

i_alpha_hat_next = i_alpha_hat_z + Ts*di_alpha_hat;
i_beta_hat_next  = i_beta_hat_z  + Ts*di_beta_hat;

% Back-EMF observer dynamics (discrete Euler)
de_alpha_hat = ke * i_alpha_tilde;
de_beta_hat  = ke * i_beta_tilde;

e_alpha_hat_next = e_alpha_hat_z + Ts*de_alpha_hat;
e_beta_hat_next  = e_beta_hat_z  + Ts*de_beta_hat;

% Optional: saturation on e_hat to avoid wind-up
E_MAX = 1e4; % set based on machine
e_alpha_hat_next = min(max(e_alpha_hat_next, -E_MAX), E_MAX);
e_beta_hat_next  = min(max(e_beta_hat_next,  -E_MAX),  E_MAX);

% Update state
i_alpha_hat_z = i_alpha_hat_next;
i_beta_hat_z  = i_beta_hat_next;
e_alpha_hat_z = e_alpha_hat_next;
e_beta_hat_z  = e_beta_hat_next;

% Outputs
i_alpha_hat = i_alpha_hat_z;
i_beta_hat  = i_beta_hat_z;
e_alpha_hat = e_alpha_hat_z;
e_beta_hat  = e_beta_hat_z;
end

== matlab function TestModel_V5_Timing_V3_2024a/Motor/MATLAB Function3 ==
  data: Vc input; Vab output; Vb input; Va input; Vbc output; Vca output
function [Vab,Vbc,Vca] = fcn(Vc,Vb,Va)
%#codegen

% if fe<6
%     Vs=Vs1+V_Boost;
% else
%     Vs=Vs1;
% end

Vab=Va-Vb;
Vbc=Vb-Vc;
Vca=Vc-Va;

end

== matlab function TestModel_V5_Timing_V3_2024a/Subsystem2/Pre_Mag_V1/MATLAB Function ==
  data: StartPulse input; PreMag_En output
function PreMag_En = PreMagState(StartPulse)

persistent timer active

Ts = 1e-6;
PreMagTime = 0.2;    % 200 ms

if isempty(timer)
    timer = 0;
    active = 0;
end

if isempty(active)
    timer = 0;
    active = 0;
end

if StartPulse
    %timer = 0;
    active = 1;
    timer = timer + Ts;
    if timer >= PreMagTime
        active = 0;
    end
end

% if active
% 
%     timer = timer + Ts;
% 
%     if timer >= PreMagTime
%         active = 0;
%     end
% 
% end

% if StartPulse
%     timer = 0;
%     active = 1;
% end
% 
% if active
% 
%     timer = timer + Ts;
% 
%     if timer >= PreMagTime
%         active = 0;
%     end
% 
% end

PreMag_En = active;
end
